simulink model "nms_sim_2D_cost"  (R2024b)
settings: Solver=ode15s  StartTime=0.0  StopTime=t_sim  MaxStep=dt_max  EnableMultiTasking=on
values from neighbouring files (symbols this model uses):
  a_BFSH = param_ctrl(35)*1    [setCtrlPar_optim_CPGreflex2001_2D.m]
  a_GAS = param_ctrl(37)*1    [setCtrlPar_optim_CPGreflex2001_2D.m]
  a_GLU = param_ctrl(31)*1    [setCtrlPar_optim_CPGreflex2001_2D.m]
  a_HAM = param_ctrl(33)*1    [setCtrlPar_optim_CPGreflex2001_2D.m]
  a_HFL = param_ctrl(32)*1    [setCtrlPar_optim_CPGreflex2001_2D.m]
  a_RF = param_ctrl(34)*1    [setCtrlPar_optim_CPGreflex2001_2D.m]
  a_SOL = param_ctrl(38)*1    [setCtrlPar_optim_CPGreflex2001_2D.m]
  a_TA = param_ctrl(39)*1    [setCtrlPar_optim_CPGreflex2001_2D.m]
  a_VAS = param_ctrl(36)*1    [setCtrlPar_optim_CPGreflex2001_2D.m]
  ai = param_ctrl(96)*2.0    [setCtrlPar_optim_CPGreflex2001_2D.m]
  b_BFSH = param_ctrl(52)*.51    [setCtrlPar_optim_CPGreflex2001_2D.m]
  b_BFSHGAS = param_ctrl(55)*.51    [setCtrlPar_optim_CPGreflex2001_2D.m]
  b_BFSHHAM = param_ctrl(54)*.51    [setCtrlPar_optim_CPGreflex2001_2D.m]
  b_BFSHVAS = param_ctrl(53)*.51    [setCtrlPar_optim_CPGreflex2001_2D.m]
  b_GAS = param_ctrl(59)*.51    [setCtrlPar_optim_CPGreflex2001_2D.m]
  b_GASBFSH = param_ctrl(60)*.51    [setCtrlPar_optim_CPGreflex2001_2D.m]
  b_GASSOL = param_ctrl(61)*.51    [setCtrlPar_optim_CPGreflex2001_2D.m]
  b_GLU = param_ctrl(40)*.51    [setCtrlPar_optim_CPGreflex2001_2D.m]
  b_GLUHAM = param_ctrl(42)*.51    [setCtrlPar_optim_CPGreflex2001_2D.m]
  b_GLUHFL = param_ctrl(41)*.51    [setCtrlPar_optim_CPGreflex2001_2D.m]
  b_HAM = param_ctrl(46)*.51    [setCtrlPar_optim_CPGreflex2001_2D.m]
  b_HAMBFSH = param_ctrl(48)*.51    [setCtrlPar_optim_CPGreflex2001_2D.m]
  b_HAMGLU = param_ctrl(47)*.51    [setCtrlPar_optim_CPGreflex2001_2D.m]
  b_HFL = param_ctrl(43)*.51    [setCtrlPar_optim_CPGreflex2001_2D.m]
  b_HFLGLU = param_ctrl(44)*.51    [setCtrlPar_optim_CPGreflex2001_2D.m]
  b_HFLRF = param_ctrl(45)*.51    [setCtrlPar_optim_CPGreflex2001_2D.m]
  b_RF = param_ctrl(49)*.51    [setCtrlPar_optim_CPGreflex2001_2D.m]
  b_RFHFL = param_ctrl(50)*.51    [setCtrlPar_optim_CPGreflex2001_2D.m]
  b_RFVAS = param_ctrl(51)*.51    [setCtrlPar_optim_CPGreflex2001_2D.m]
  b_SOL = param_ctrl(62)*.51    [setCtrlPar_optim_CPGreflex2001_2D.m]
  b_SOLGAS = param_ctrl(64)*.51    [setCtrlPar_optim_CPGreflex2001_2D.m]
  b_SOLTA = param_ctrl(63)*.51    [setCtrlPar_optim_CPGreflex2001_2D.m]
  b_TA = param_ctrl(65)*.51    [setCtrlPar_optim_CPGreflex2001_2D.m]
  b_TASOL = param_ctrl(66)*.51    [setCtrlPar_optim_CPGreflex2001_2D.m]
  b_VAS = param_ctrl(56)*.51    [setCtrlPar_optim_CPGreflex2001_2D.m]
  b_VASBFSH = param_ctrl(57)*.51    [setCtrlPar_optim_CPGreflex2001_2D.m]
  b_VASRF = param_ctrl(58)*.51    [setCtrlPar_optim_CPGreflex2001_2D.m]
  bias = param_ctrl(97)*2.5    [setCtrlPar_optim_CPGreflex2001_2D.m]
  c = 0.05    [nms_MS_2D_scaled.m]
  c_jointstop = 0.3 / (pi/180)    (= 17.1887338539)    [nms_MS_2D_scaled.m]
  D12_F = 0.16    *scaleL_JPhys    [nms_MechInit_2D_scaleSkel.m]
  D12_S = 0.2460	*sub_height    [nms_MechInit_2D_scaleSkel.m]
  D12_T = 0.2450  *sub_height    [nms_MechInit_2D_scaleSkel.m]
  D12y_F = 0.039  *sub_height    [nms_MechInit_2D_scaleSkel.m]
  D12z_HAT = 0.1    [nms_MS_2D_scaled.m]
  D13_F = 0.20    *scaleL_JPhys    [nms_MechInit_2D_scaleSkel.m]
  D1G_F = 0.14    *scaleL_JPhys    [nms_MechInit_2D_scaleSkel.m]
  D1G_HAT = 0.35  *scaleL_JPhys    [nms_MechInit_2D_scaleSkel.m]
  D1G_S = (0.3 - D12y_F/4)	*scaleL_JPhys    [nms_MechInit_2D_scaleSkel.m]
  D1G_T = (0.3 - D12y_F/4)	*scaleL_JPhys    [nms_MechInit_2D_scaleSkel.m]
  D1Gy_F = D12y_F*D1G_F/D12_F    (= 0.07)    [nms_MechInit_2D_scaleSkel.m]
  d_BFSH = param_ctrl(26)*1    [setCtrlPar_optim_CPGreflex2001_2D.m]
  d_GAS = param_ctrl(28)*1    [setCtrlPar_optim_CPGreflex2001_2D.m]
  d_GLU = param_ctrl(22)*1    [setCtrlPar_optim_CPGreflex2001_2D.m]
  d_HAM = param_ctrl(24)*1    [setCtrlPar_optim_CPGreflex2001_2D.m]
  d_HFL = param_ctrl(23)*1    [setCtrlPar_optim_CPGreflex2001_2D.m]
  d_RF = param_ctrl(25)*1    [setCtrlPar_optim_CPGreflex2001_2D.m]
  d_SOL = param_ctrl(29)*1    [setCtrlPar_optim_CPGreflex2001_2D.m]
  d_TA = param_ctrl(30)*1    [setCtrlPar_optim_CPGreflex2001_2D.m]
  d_VAS = param_ctrl(27)*1    [setCtrlPar_optim_CPGreflex2001_2D.m]
  DeltaThRef = 5e-3    (= 0.005)    [nms_MS_2D_scaled.m]
  dloptBFSH = 3.0    (= 3)    [setCtrlPar_optim_CPGreflex2001_2D.m]
  dloptGAS = 3.0    (= 3)    [setCtrlPar_optim_CPGreflex2001_2D.m]
  dloptGLU = 3.0    (= 3)    [setCtrlPar_optim_CPGreflex2001_2D.m]
  dloptHAM = 3.0    (= 3)    [setCtrlPar_optim_CPGreflex2001_2D.m]
  dloptHFL = 3.0    (= 3)    [setCtrlPar_optim_CPGreflex2001_2D.m]
  dloptRF = 3.0    (= 3)    [setCtrlPar_optim_CPGreflex2001_2D.m]
  dloptSOL = 3.0    (= 3)    [setCtrlPar_optim_CPGreflex2001_2D.m]
  dloptTA = 3.0    (= 3)    [setCtrlPar_optim_CPGreflex2001_2D.m]
  dloptVAS = 3.0    (= 3)    [setCtrlPar_optim_CPGreflex2001_2D.m]
  ec_BFSH = param_ctrl(80)*0.15    [setCtrlPar_optim_CPGreflex2001_2D.m]
  ec_GAS = param_ctrl(82)*0.15    [setCtrlPar_optim_CPGreflex2001_2D.m]
  ec_GLU = param_ctrl(76)*0.15    [setCtrlPar_optim_CPGreflex2001_2D.m]
  ec_HAM = param_ctrl(78)*0.15    [setCtrlPar_optim_CPGreflex2001_2D.m]
  ec_HFL = param_ctrl(77)*0.15    [setCtrlPar_optim_CPGreflex2001_2D.m]
  ec_RF = param_ctrl(79)*0.15    [setCtrlPar_optim_CPGreflex2001_2D.m]
  ec_TA = param_ctrl(84)*0.15    [setCtrlPar_optim_CPGreflex2001_2D.m]
  ec_VAS = param_ctrl(81)*0.15    [setCtrlPar_optim_CPGreflex2001_2D.m]
  eref = 0.04    [nms_MS_2D_scaled.m]
  eref_GAS = 0.1    [nms_MS_2D_scaled.m]
  eref_SOL = 0.1    [nms_MS_2D_scaled.m]
  es_BFSH = param_ctrl(89)*0.15    [setCtrlPar_optim_CPGreflex2001_2D.m]
  es_GAS = param_ctrl(91)*0.15    [setCtrlPar_optim_CPGreflex2001_2D.m]
  es_GLU = param_ctrl(85)*0.15    [setCtrlPar_optim_CPGreflex2001_2D.m]
  es_HAM = param_ctrl(87)*0.15    [setCtrlPar_optim_CPGreflex2001_2D.m]
  es_HFL = param_ctrl(86)*0.15    [setCtrlPar_optim_CPGreflex2001_2D.m]
  es_RF = param_ctrl(88)*0.15    [setCtrlPar_optim_CPGreflex2001_2D.m]
  es_TA = param_ctrl(93)*0.15    [setCtrlPar_optim_CPGreflex2001_2D.m]
  es_VAS = param_ctrl(90)*0.15    [setCtrlPar_optim_CPGreflex2001_2D.m]
  FmaxBFSH = 350    [nms_MS_2D_scaled.m]
  FmaxGAS = 2000    [nms_MS_2D_scaled.m]
  FmaxGLU = 4000    [nms_MS_2D_scaled.m]
  FmaxHAM = 2000    [nms_MS_2D_scaled.m]
  FmaxHFL = 2000    [nms_MS_2D_scaled.m]
  FmaxRF = 850    [nms_MS_2D_scaled.m]
  FmaxSOL = 4000    [nms_MS_2D_scaled.m]
  FmaxTA = 800    [nms_MS_2D_scaled.m]
  FmaxVAS = 5000    [nms_MS_2D_scaled.m]
  g = 9.81    [nms_MS_2D_scaled.m]
  gamma_4 = param_ctrl(11) * 1.7    [setCtrlPar_optim_CPGreflexsynergy2023_2D.m]
  h_BFSH = param_ctrl(71)*.1    [setCtrlPar_optim_CPGreflex2001_2D.m]
  h_GAS = param_ctrl(73)*.1    [setCtrlPar_optim_CPGreflex2001_2D.m]
  h_GLU = param_ctrl(67)*.1    [setCtrlPar_optim_CPGreflex2001_2D.m]
  h_HAM = param_ctrl(69)*.1    [setCtrlPar_optim_CPGreflex2001_2D.m]
  h_HFL = param_ctrl(68)*.1    [setCtrlPar_optim_CPGreflex2001_2D.m]
  h_RF = param_ctrl(70)*.1    [setCtrlPar_optim_CPGreflex2001_2D.m]
  h_SOL = param_ctrl(74)*.1    [setCtrlPar_optim_CPGreflex2001_2D.m]
  h_TA = param_ctrl(75)*.1    [setCtrlPar_optim_CPGreflex2001_2D.m]
  h_VAS = param_ctrl(72)*.1    [setCtrlPar_optim_CPGreflex2001_2D.m]
  HLCtrlPar = [theta_tgt l_clr alpha_tgt alpha_cd alpha_cv]    [setCtrlPar_optim_reflex2015_2D.m]
  In_F = 0.005    *scaleM*scaleL_JPhys^2    [nms_MechInit_2D_scaleSkel.m]
  In_HAT = 2.5    *scaleM*scaleL_JPhys^2    [nms_MechInit_2D_scaleSkel.m]
  In_S = 0.05     *scaleM*scaleL_JPhys^2    [nms_MechInit_2D_scaleSkel.m]
  In_T = 0.15     *scaleM*scaleL_JPhys^2    [nms_MechInit_2D_scaleSkel.m]
  init_exc = 0.01    [setInitPar_optim_2D.m]
  init_fm = 0.01    [setInitPar_optim_2D.m]
  init_lce = 1    [setInitPar_optim_2D.m]
  init_LCPG = param_ctrl(12) * 0.01    [setCtrlPar_optim_CPGreflexsynergy2023_2D.m]
  init_LStance = 1    [setInitPar_optim_2D.m]
  init_N1 = osc_signal1(phi_off_osc_ind)    [setCtrlPar_optim_CPGreflex2001_2D.m]
  ... (+441 more)
undefined symbols (not defined in the file or in its folder): cost_act_exponent, cost_v_tgt, flag_controller, Newton, nStep_obj, nStep_startKin, Raphson, sgn, SSW_kin, terrain_slope_angle, v_plateS1, X, Y, Z
libraries: nesl_utility x94, sm_lib x90, simulink x28, simulink_extras x12
(part 3 of 20)

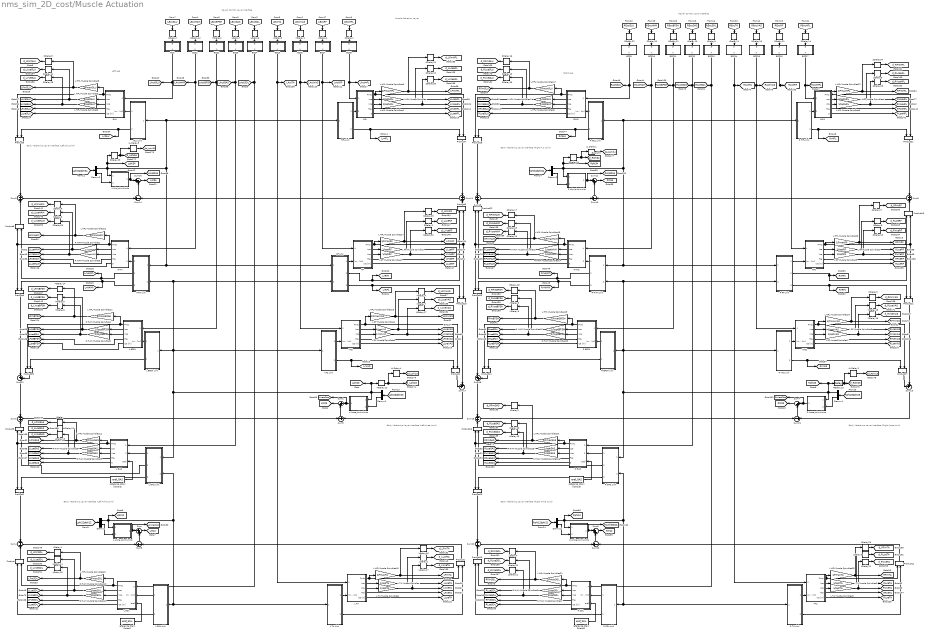
== system nms_sim_2D_cost/Muscle Actuation ==
  note: Left Leg
  note: Neural Control Layer Interface
  note: Muscle Actuation Layer
  note: Body Mechanics Layer
      | Interface (Left Hip Joint)
  note: Body Mechanics Layer
      | Interface (Left Knee Joint)
  note: Body Mechanics Layer
      | Interface (Left Ankle Joint)
  note: Right Leg
  note: Neural Control Layer Interface
  note: Body Mechanics Layer
      | Interface (Right Hip Joint)
  note: Body Mechanics Layer
      | Interface (Right Knee Joint)
  note: Body Mechanics Layer
      | Interface (Right Ankle Joint)
  Demux{,1..5} (6 alike) : Demux  Outputs=2
  ECC : Subsystem
  ECC1 : Subsystem
  ECC10 : Subsystem
  ECC11 : Subsystem
  ECC12 : Subsystem
  ECC13 : Subsystem
  ECC14 : Subsystem
  ECC15 : Subsystem
  ECC16 : Subsystem
  ECC17 : Subsystem
  ECC2 : Subsystem
  ECC3 : Subsystem
  ECC4 : Subsystem
  ECC5 : Subsystem
  ECC6 : Subsystem
  ECC7 : Subsystem
  ECC8 : Subsystem
  ECC9 : Subsystem
  GLU : Subsystem
  GLU Link : Subsystem
  GLU1 : Subsystem
  HAM : Subsystem
  HAM Link : Subsystem
  HAM1 : Subsystem
  HFL : Subsystem
  HFL Link : Subsystem
  HFL1 : Subsystem
  L Ankle Joint Limits : Subsystem
  L BFSH : Subsystem
  L BFSH Link : Subsystem
  L GAS : Subsystem
  L GAS Link : Subsystem
  L HFL Muscle Spindles{,1,4..5} (4 alike) : Gain  Gain=1/loptHFL
  L HFL Muscle Spindles10 : Gain  Gain=1/FmaxHAM
  L HFL Muscle Spindles11 : Gain  Gain=1/FmaxBFSH
  L HFL Muscle Spindles12 : Gain  Gain=1/FmaxGAS
  L HFL Muscle Spindles13 : Gain  Gain=1/FmaxSOL
  L HFL Muscle Spindles14 : Gain  Gain=1/FmaxRF
  L HFL Muscle Spindles15 : Gain  Gain=1/FmaxVAS
  L HFL Muscle Spindles16 : Gain  Gain=1/FmaxTA
  L HFL Muscle Spindles17 : Gain  Gain=1/FmaxGLU
  L HFL Muscle Spindles18 : Gain  Gain=1/FmaxHAM
  L HFL Muscle Spindles19 : Gain  Gain=1/FmaxBFSH
  L HFL Muscle Spindles{2..3,6..7} (4 alike) : Gain  Gain=1/loptGLU
  L HFL Muscle Spindles20 : Gain  Gain=1/FmaxGAS
  L HFL Muscle Spindles21 : Gain  Gain=1/FmaxSOL
  L HFL Muscle Spindles22 : Gain  Gain=1/FmaxHFL
  L HFL Muscle Spindles23 : Gain  Gain=1/FmaxRF
  L HFL Muscle Spindles24 : Gain  Gain=1/FmaxVAS
  L HFL Muscle Spindles25 : Gain  Gain=1/FmaxTA
  L HFL Muscle Spindles8 : Gain  Gain=1/FmaxGLU
  L HFL Muscle Spindles9 : Gain  Gain=1/FmaxHFL
  L Hip Joint Limits : Subsystem
  L Knee Joint Limits : Subsystem
  L RF Muscle Spindles{,1..3} (4 alike) : Gain  Gain=1/loptRF
  L RF Muscle Spindles{4..7} (4 alike) : Gain  Gain=1/loptVAS
  L SOL : Subsystem
  L SOL Link : Subsystem
  L TA : Subsystem
  L TA Muscle Spindles{,1..3} (4 alike) : Gain  Gain=1/loptTA
  L TA Link : Subsystem
  LDelay{,1,3..4,16,23} (6 alike) : TransportDelay  DelayTime=LongDelay  InitialOutput=init_fm
  LDelay{6..11} (6 alike) : TransportDelay  DelayTime=LongDelay  InitialOutput=init_exc
  LDelay{2,5,12,14,18,20} (6 alike) : TransportDelay  DelayTime=LongDelay  InitialOutput=init_lce
  LDelay{13,15,17,19,21..22} (6 alike) : TransportDelay  DelayTime=LongDelay  InitialOutput=init_vce
  LL Delay{1..4} (4 alike) : TransportDelay  DelayTime=LongLoopDelay
  MDelay{1..2,10..11} (4 alike) : TransportDelay  DelayTime=MidDelay  InitialOutput=init_exc
  MDelay12 : TransportDelay  DelayTime=MidDelay  InitialOutput=Lphi230
  MDelay13 : TransportDelay  DelayTime=MidDelay  InitialOutput=Lphi230
  MDelay{3..4,14,18} (4 alike) : TransportDelay  DelayTime=MidDelay  InitialOutput=init_fm
  MDelay{5,7..8,15} (4 alike) : TransportDelay  DelayTime=MidDelay  InitialOutput=init_lce
  MDelay{6,9,16..17} (4 alike) : TransportDelay  DelayTime=MidDelay  InitialOutput=init_vce
  Product{,1..23} (24 alike) : Product  RndMeth=Zero
  R Ankle Joint Limits : Subsystem
  R BFSH : Subsystem
  R BFSH Link : Subsystem
  R GAS : Subsystem
  R GAS Link : Subsystem
  R GLU Link : Subsystem
  R HAM Muscle Spindles{1,3,6,14} (4 alike) : Gain  Gain=1/loptHAM
  R HAM Muscle Spindles{5,7,10..11} (4 alike) : Gain  Gain=1/loptSOL
  R HAM Muscle Spindles{2,4,12..13} (4 alike) : Gain  Gain=1/loptBFSH
  R HAM Muscle Spindles{8..9,15..16} (4 alike) : Gain  Gain=1/loptGAS
  R HAM Link : Subsystem
  R HFL Link : Subsystem
  R Hip Joint Limits : Subsystem
  R Knee Joint Limits : Subsystem
  R RF Link : Subsystem
  R SOL : Subsystem
  R SOL Link : Subsystem
  R TA Link : Subsystem
  R VAS Link : Subsystem
  RF : Subsystem
  RF Link : Subsystem
  RF1 : Subsystem
  SDelay{1,4,7,12,14,20..22} (8 alike) : TransportDelay  DelayTime=ShortDelay  InitialOutput=init_exc
  SDelay{2..3,5..6,10..11,13,15} (8 alike) : TransportDelay  DelayTime=ShortDelay  InitialOutput=init_lce
  SDelay{8..9,16..17,27,29,31,34} (8 alike) : TransportDelay  DelayTime=ShortDelay  InitialOutput=init_fm
  SDelay{18..19,25..26,28,30,32..33} (8 alike) : TransportDelay  DelayTime=ShortDelay  InitialOutput=init_vce
  SDelay23 : TransportDelay  DelayTime=ShortDelay  InitialOutput=Lphi340
  SDelay24 : TransportDelay  DelayTime=ShortDelay  InitialOutput=Lphi340
  Sum{,1,6..7,12,16,18,22} (8 alike) : Sum  Inputs=|++
  Sum{9..10,14,23} (4 alike) : Sum  Inputs=+-
  Sum{2..4,8,11,15,19..20} (8 alike) : Sum
  Sum13 : Sum  Inputs=++|
  Sum17 : Sum  Inputs=++|
  Sum21 : Sum  Inputs=-+
  Sum5 : Sum  Inputs=-+
  TA1 : Subsystem
  VAS : Subsystem
  VAS Link : Subsystem
  VAS1 : Subsystem
  reference strain [lslack] : Constant  Value=eref_SOL
  reference strain [lslack]1 : Constant  Value=eref_SOL
  reference strain [lslack]2 : Constant  Value=eref_GAS
  reference strain [lslack]3 : Constant  Value=eref_GAS
  tag scope: LActBFSH=global, LActGAS=global, LActGLU=global, LActHAM=global, LActHFL=global, LActRF=global, LActSOL=global, LActTA=global, LActVAS=global, LAnkleStop=global, LFceBFSH=global, LFceGAS=global, LFceGLU=global, LFceHAM=global, LFceHFL=global, LFceRF=global, LFceSOL=global, LFceTA=global, LFceVAS=global, LFmBFSH=global, LFmGAS=global, LFmGLU=global, LFmHAM=global, LFmHFL=global, LFmRF=global, LFmSOL=global, LFmTA=global, LFmVAS=global, LHipStop=global, LKneeStop=global, LLceBFSH=global, LLceGAS=global, LLceGLU=global, LLceHAM=global, LLceHFL=global, LLceRF=global, LLceSOL=global, LLceTA=global, LLceVAS=global, LLseBFSH=global, LLseGAS=global, LLseGLU=global, LLseHAM=global, LLseHFL=global, LLseRF=global, LLseSOL=global, LLseTA=global, LLseVAS=global, LM12=global, LM23=global, LM34=global, LVceBFSH=global, LVceGAS=global, LVceGLU=global, LVceHAM=global, LVceHFL=global, LVceRF=global, LVceSOL=global, LVceTA=global, LVceVAS=global, Lphi12=global, Lphi23=global, Lphi34=global, LrGLU=global, LrHAMh=global, LrHAMk=global, LrHFL=global, LrRFh=global, LrRFk=global, LrVAS=global, RActBFSH=global, RActGAS=global, RActGLU=global, RActHAM=global, RActHFL=global, RActRF=global, RActSOL=global, RActTA=global, RActVAS=global, RAnkleStop=global, RFceBFSH=global, RFceGAS=global, RFceGLU=global, RFceHAM=global, RFceHFL=global, RFceRF=global, RFceSOL=global, RFceTA=global, RFceVAS=global, RFmBFSH=global, RFmGAS=global, RFmGLU=global, RFmHAM=global, RFmHFL=global, RFmRF=global, RFmSOL=global, RFmTA=global, RFmVAS=global, RHipStop=global, RKneeStop=global, RLceBFSH=global, RLceGAS=global, RLceGLU=global, RLceHAM=global, RLceHFL=global, RLceRF=global, RLceSOL=global, RLceTA=global, RLceVAS=global, RLseBFSH=global, RLseGAS=global, RLseGLU=global, RLseHAM=global, RLseHFL=global, RLseRF=global, RLseSOL=global, RLseTA=global, RLseVAS=global, RM12=global, RM23=global, RM34=global, RVceBFSH=global, RVceGAS=global, RVceGLU=global, RVceHAM=global, RVceHFL=global, RVceRF=global, RVceSOL=global, RVceTA=global, RVceVAS=global, Rphi12=global, Rphi23=global, Rphi34=global, RrGLU=global, RrHAMh=global, RrHAMk=global, RrHFL=global, RrRFh=global, RrRFk=global, RrVAS=global, d_LFmBFSH=global, d_LFmGAS=global, d_LFmGLU=global, d_LFmHAM=global, d_LFmHFL=global, d_LFmRF=global, d_LFmSOL=global, d_LFmTA=global, d_LFmVAS=global, d_LLceBFSH=global, d_LLceGAS=global, d_LLceGLU=global, d_LLceHAM=global, d_LLceHFL=global, d_LLceRF=global, d_LLceSOL=global, d_LLceTA=global, d_LLceVAS=global, d_LVceBFSH=global, d_LVceGAS=global, d_LVceGLU=global, d_LVceHAM=global, d_LVceHFL=global, d_LVceRF=global, d_LVceSOL=global, d_LVceTA=global, d_LVceVAS=global, d_Lphi23=global, d_Lphi34=global, d_RFmBFSH=global, d_RFmGAS=global, d_RFmGLU=global, d_RFmHAM=global, d_RFmHFL=global, d_RFmRF=global, d_RFmSOL=global, d_RFmTA=global, d_RFmVAS=global, d_RLceBFSH=global, d_RLceGAS=global, d_RLceGLU=global, d_RLceHAM=global, d_RLceHFL=global, d_RLceRF=global, d_RLceSOL=global, d_RLceTA=global, d_RLceVAS=global, d_RVceBFSH=global, d_RVceGAS=global, d_RVceGLU=global, d_RVceHAM=global, d_RVceHFL=global, d_RVceRF=global, d_RVceSOL=global, d_RVceTA=global, d_RVceVAS=global, d_Rphi23=global, d_Rphi34=global, dd_Lphi23=global, dd_Lphi34=global, dd_Rphi23=global, dd_Rphi34=global
  wires:
  Demux1/1 -> L Knee Joint Limits/1(phi [rad]), L BFSH Link/1(phi23 [rad]), HAM Link/2(phi23 [rad]), RF Link/2(phi23 [rad]), VAS Link/1(phi23 [rad]), L GAS Link/1(phi23 [rad]), MDelay12/1, [Lphi23]
  L SOL/1(Fmtc) -> L HFL Muscle Spindles13/1, Product/2
  L TA/2(Lce) -> L TA Muscle Spindles/1
  L GAS/1(Fmtc) -> Product2/1, Product3/1, L HFL Muscle Spindles12/1
  Demux/1 -> L SOL Link/1(phi12 [rad]), L TA Link/1(phi12 [rad]), L GAS Link/2(phi12 [rad]), L Ankle Joint Limits/1(phi [rad]), [Lphi12]
  HAM/1(Fmtc) -> Product9/1, Product8/1, L HFL Muscle Spindles10/1
  HAM/2(Lce) -> R HAM Muscle Spindles1/1
  HFL/1(Fmtc) -> L HFL Muscle Spindles9/1, Product7/2
  HFL/2(Lce) -> L HFL Muscle Spindles/1
  GLU/1(Fmtc) -> Product6/1, L HFL Muscle Spindles8/1
  Sum16/1 -> [LM34]
  Demux/2 -> L Ankle Joint Limits/2(dphi [rad/s])
  Sum9/1 -> Sum/2
  Demux1/2 -> L Knee Joint Limits/2(dphi [rad/s])
  L SOL Link/1(lmtc [m]) -> L SOL/2(lmtc [m])
  L TA Link/1(lmtc [m]) -> L TA/2(lmtc [m])
  L GAS Link/3(lever12 [m]) -> Product2/2
  L GAS Link/2(lever23 [m]) -> Product3/2
  L GAS Link/1(lmtu [m]) -> L GAS/2(lmtc [m])
  VAS Link/1(lmtu [m]) -> VAS/2(lmtc [m])
  HAM Link/1(lmtu [m]) -> HAM/2(lmtc [m])
  HAM Link/2(lever34 [m]) -> Product8/2, [LrHAMh]
  HAM Link/3(lever23 [m]) -> Product9/2, [LrHAMk]
  Product3/1 -> Sum2/2
  Sum3/1 -> Sum14/1
  Sum4/1 -> Sum9/1
  [Lphi12dphi12] -> Demux/1
  [Lphi23dphi23] -> Demux1/1
  [Lphi34dphi34] -> Demux2/1
  Demux2/1 -> L Hip Joint Limits/1(phi [rad]), HFL Link/1(phi34 [rad]), GLU Link/1(phi34 [rad]), RF Link/1(phi34 [rad]), HAM Link/1(phi34 [rad]), [Lphi34], SDelay23/1
  L SOL Link/2(lever [m]) -> Product/1
  Product/1 -> Sum4/2
  Product2/1 -> Sum4/1
  L TA Link/2(lever [m]) -> Product1/2
  Product1/1 -> Sum9/2
  L Ankle Joint Limits/1(M_stop [Nm]) -> Sum/1, [LAnkleStop]
  Sum/1 -> [LM12]
  VAS/1(Fmtc) -> Product4/2, L HFL Muscle Spindles15/1
  Sum1/1 -> [LM23]
  L Knee Joint Limits/1(M_stop [Nm]) -> Sum1/1, [LKneeStop]
  Sum5/1 -> Sum1/2
  VAS Link/2(lever [m]) -> [LrVAS], Product4/1
  Sum2/1 -> Sum5/1
  Product8/1 -> Sum3/2
  Product6/1 -> Sum3/1
  GLU Link/1(lmtu [m]) -> GLU/2(lmtc [m])
  GLU Link/2(lever [m]) -> [LrGLU], Product6/2
  Demux2/2 -> L Hip Joint Limits/2(dphi [rad/s])
  L Hip Joint Limits/1(M_stop [Nm]) -> Sum16/1, [LHipStop]
  Sum14/1 -> Sum16/2
  HFL Link/1(lmtu [m]) -> HFL/2(lmtc [m])
  HFL Link/2(lever [m]) -> Product7/1, [LrHFL]
  GLU/2(Lce) -> L HFL Muscle Spindles3/1
  GLU/3(Vce) -> L HFL Muscle Spindles2/1
  HAM/3(Vce) -> R HAM Muscle Spindles6/1
  L GAS/3(Vce) -> R HAM Muscle Spindles9/1
  L GAS/2(Lce) -> R HAM Muscle Spindles8/1
  L SOL/2(Lce) -> R HAM Muscle Spindles10/1
  L SOL/3(Vce) -> R HAM Muscle Spindles11/1
  L TA/3(Vce) -> L TA Muscle Spindles1/1
  VAS/3(Vce) -> L RF Muscle Spindles6/1
  VAS/2(Lce) -> L RF Muscle Spindles4/1
  HFL/3(Vce) -> L HFL Muscle Spindles1/1
  RF/3(Vce) -> L RF Muscle Spindles2/1
  RF/2(Lce) -> L RF Muscle Spindles/1
  RF Link/1(lmtu [m]) -> RF/2(lmtc [m])
  RF Link/2(lever34 [m]) -> Product5/1, [LrRFh]
  RF Link/3(lever23 [m]) -> Product15/1, [LrRFk]
  Product7/1 -> Sum11/1
  Product5/1 -> Sum11/2
  Product15/1 -> Sum17/2
  Sum17/1 -> Sum5/2
  Product4/1 -> Sum17/1
  L BFSH Link/1(lmtu [m]) -> L BFSH/2(lmtc [m])
  L BFSH Link/2(lever [m]) -> Product20/2
  L BFSH/2(Lce) -> R HAM Muscle Spindles4/1
  L BFSH/3(Vce) -> R HAM Muscle Spindles2/1
  Product20/1 -> Sum22/2
  Sum22/1 -> Sum2/1
  Product9/1 -> Sum22/1
  L HFL Muscle Spindles1/1 -> SDelay30/1, [LVceHFL]
  L HFL Muscle Spindles2/1 -> SDelay25/1, [LVceGLU]
  L HFL Muscle Spindles3/1 -> SDelay11/1, [LLceGLU]
  L RF Muscle Spindles6/1 -> [LVceVAS], MDelay17/1
  RF/1(Fmtc) -> Product15/2, Product5/2, L HFL Muscle Spindles14/1
  L BFSH/1(Fmtc) -> Product20/1, L HFL Muscle Spindles11/1
  R HAM Muscle Spindles8/1 -> LDelay12/1, [LLceGAS]
  R HAM Muscle Spindles9/1 -> LDelay13/1, [LVceGAS]
  R HAM Muscle Spindles10/1 -> LDelay14/1, [LLceSOL]
  R HAM Muscle Spindles11/1 -> LDelay15/1, [LVceSOL]
  L TA/1(Fmtc) -> Product1/1, L HFL Muscle Spindles16/1
  L TA Muscle Spindles1/1 -> LDelay17/1, [LVceTA]
  L HFL Muscle Spindles/1 -> SDelay10/1, [LLceHFL]
  R HAM Muscle Spindles1/1 -> SDelay3/1, [LLceHAM]
  R HAM Muscle Spindles6/1 -> SDelay33/1, [LVceHAM]
  L RF Muscle Spindles/1 -> SDelay2/1, [LLceRF]
  L RF Muscle Spindles2/1 -> SDelay32/1, [LVceRF]
  R HAM Muscle Spindles4/1 -> MDelay5/1, [LLceBFSH]
  R HAM Muscle Spindles2/1 -> MDelay6/1, [LVceBFSH]
  L RF Muscle Spindles4/1 -> [LLceVAS], MDelay7/1
  L TA Muscle Spindles/1 -> [LLceTA], LDelay2/1
  Demux4/1 -> R Knee Joint Limits/1(phi [rad]), R VAS Link/1(phi23 [rad]), R RF Link/2(phi23 [rad]), R HAM Link/2(phi23 [rad]), R BFSH Link/1(phi23 [rad]), R GAS Link/1(phi23 [rad]), MDelay13/1, [Rphi23]
  R SOL/1(Fmtc) -> Product10/2, L HFL Muscle Spindles21/1
  TA1/2(Lce) -> L TA Muscle Spindles2/1
  R GAS/1(Fmtc) -> Product13/1, Product16/1, L HFL Muscle Spindles20/1
  Demux3/1 -> R SOL Link/1(phi12 [rad]), R TA Link/1(phi12 [rad]), R GAS Link/2(phi12 [rad]), R Ankle Joint Limits/1(phi [rad]), [Rphi12]
  HAM1/1(Fmtc) -> Product23/1, Product22/1, L HFL Muscle Spindles18/1
  HAM1/2(Lce) -> R HAM Muscle Spindles3/1
  HFL1/1(Fmtc) -> L HFL Muscle Spindles22/1, Product21/2
  HFL1/2(Lce) -> L HFL Muscle Spindles4/1
  GLU1/1(Fmtc) -> Product19/1, L HFL Muscle Spindles17/1
  Sum12/1 -> [RM34]
  Demux3/2 -> R Ankle Joint Limits/2(dphi [rad/s])
  Sum23/1 -> Sum6/2
  Demux4/2 -> R Knee Joint Limits/2(dphi [rad/s])
  R SOL Link/1(lmtc [m]) -> R SOL/2(lmtc [m])
  R TA Link/1(lmtc [m]) -> TA1/2(lmtc [m])
  R GAS Link/3(lever12 [m]) -> Product13/2
  R GAS Link/2(lever23 [m]) -> Product16/2
  R GAS Link/1(lmtu [m]) -> R GAS/2(lmtc [m])
  R HAM Link/1(lmtu [m]) -> HAM1/2(lmtc [m])
  R HAM Link/2(lever34 [m]) -> Product22/2, [RrHAMh]
  R HAM Link/3(lever23 [m]) -> Product23/2, [RrHAMk]
  Product16/1 -> Sum15/2
  Sum19/1 -> Sum10/1
  Sum20/1 -> Sum23/1
  [Rphi12dphi12] -> Demux3/1
  [Rphi23dphi23] -> Demux4/1
  [Rphi34dphi34] -> Demux5/1
  Demux5/1 -> R Hip Joint Limits/1(phi [rad]), R HFL Link/1(phi34 [rad]), R GLU Link/1(phi34 [rad]), R RF Link/1(phi34 [rad]), R HAM Link/1(phi34 [rad]), SDelay24/1, [Rphi34]
  R SOL Link/2(lever [m]) -> Product10/1
  Product10/1 -> Sum20/2
  Product13/1 -> Sum20/1
  R TA Link/2(lever [m]) -> Product11/2
  Product11/1 -> Sum23/2
  R Ankle Joint Limits/1(M_stop [Nm]) -> Sum6/1, [RAnkleStop]
  Sum6/1 -> [RM12]
  VAS1/1(Fmtc) -> Product17/2, L HFL Muscle Spindles24/1
  Sum7/1 -> [RM23]
  R Knee Joint Limits/1(M_stop [Nm]) -> Sum7/1, [RKneeStop]
  Sum21/1 -> Sum7/2
  R VAS Link/2(lever [m]) -> [RrVAS], Product17/1
  Sum15/1 -> Sum21/1
  Product22/1 -> Sum19/2
  Product19/1 -> Sum19/1
  R GLU Link/1(lmtu [m]) -> GLU1/2(lmtc [m])
  R GLU Link/2(lever [m]) -> Product19/2, [RrGLU]
  Demux5/2 -> R Hip Joint Limits/2(dphi [rad/s])
  R Hip Joint Limits/1(M_stop [Nm]) -> [RHipStop], Sum12/1
  Sum10/1 -> Sum12/2
  R HFL Link/1(lmtu [m]) -> HFL1/2(lmtc [m])
  R HFL Link/2(lever [m]) -> Product21/1, [RrHFL]
  GLU1/2(Lce) -> L HFL Muscle Spindles7/1
  GLU1/3(Vce) -> L HFL Muscle Spindles6/1
  HAM1/3(Vce) -> R HAM Muscle Spindles14/1
  R GAS/3(Vce) -> R HAM Muscle Spindles16/1
  R GAS/2(Lce) -> R HAM Muscle Spindles15/1
  R SOL/2(Lce) -> R HAM Muscle Spindles5/1
  R SOL/3(Vce) -> R HAM Muscle Spindles7/1
  TA1/3(Vce) -> L TA Muscle Spindles3/1
  VAS1/3(Vce) -> L RF Muscle Spindles7/1
  VAS1/2(Lce) -> L RF Muscle Spindles5/1
  HFL1/3(Vce) -> L HFL Muscle Spindles5/1
  RF1/3(Vce) -> L RF Muscle Spindles3/1
  RF1/2(Lce) -> L RF Muscle Spindles1/1
  R RF Link/2(lever34 [m]) -> Product18/1, [RrRFh]
  R RF Link/3(lever23 [m]) -> Product12/1, [RrRFk]
  Sum8/1 -> Sum10/2
  Product21/1 -> Sum8/1
  Product18/1 -> Sum8/2
  Product12/1 -> Sum13/2
  Sum13/1 -> Sum21/2
  Product17/1 -> Sum13/1
  R BFSH Link/1(lmtu [m]) -> R BFSH/2(lmtc [m])
  R BFSH Link/2(lever [m]) -> Product14/2
  R BFSH/2(Lce) -> R HAM Muscle Spindles13/1
  R BFSH/3(Vce) -> R HAM Muscle Spindles12/1
  Product14/1 -> Sum18/2
  Sum18/1 -> Sum15/1
  Product23/1 -> Sum18/1
  L HFL Muscle Spindles5/1 -> [RVceHFL], SDelay28/1
  L HFL Muscle Spindles6/1 -> SDelay26/1, [RVceGLU]
  L HFL Muscle Spindles7/1 -> SDelay13/1, [RLceGLU]
  RF1/1(Fmtc) -> Product18/2, Product12/2, L HFL Muscle Spindles23/1
  R BFSH/1(Fmtc) -> Product14/1, L HFL Muscle Spindles19/1
  R HAM Muscle Spindles15/1 -> LDelay18/1, [RLceGAS]
  R HAM Muscle Spindles16/1 -> LDelay19/1, [RVceGAS]
  R HAM Muscle Spindles5/1 -> LDelay20/1, [RLceSOL]
  R HAM Muscle Spindles7/1 -> LDelay21/1, [RVceSOL]
  TA1/1(Fmtc) -> Product11/1, L HFL Muscle Spindles25/1
  L TA Muscle Spindles3/1 -> [RVceTA], LDelay22/1
  L HFL Muscle Spindles4/1 -> [RLceHFL], SDelay6/1
  R HAM Muscle Spindles3/1 -> SDelay15/1, [RLceHAM]
  R HAM Muscle Spindles14/1 -> SDelay19/1, [RVceHAM]
  L RF Muscle Spindles1/1 -> SDelay5/1, [RLceRF]
  L RF Muscle Spindles3/1 -> SDelay18/1, [RVceRF]
  R HAM Muscle Spindles13/1 -> MDelay8/1, [RLceBFSH]
  R HAM Muscle Spindles12/1 -> MDelay9/1, [RVceBFSH]
  L RF Muscle Spindles5/1 -> MDelay15/1, [RLceVAS]
  L TA Muscle Spindles2/1 -> [RLceTA], LDelay5/1
  R VAS Link/1(lmtu [m]) -> VAS1/2(lmtc [m])
  R RF Link/1(lmtu [m]) -> RF1/2(lmtc [m])
  ECC/1(A) -> GLU/1(A), [LActGLU]
  GLU/4(Fce) -> [LFceGLU]
  GLU/5(lse [m]) -> [LLseGLU]
  L HFL Muscle Spindles10/1 -> SDelay9/1, [LFmHAM]
  ECC1/1(A) -> [LActHAM], HAM/1(A)
  HAM/4(Fce) -> [LFceHAM]
  HAM/5(lse [m]) -> [LLseHAM]
  L HFL Muscle Spindles11/1 -> MDelay14/1, [LFmBFSH]
  ECC2/1(A) -> [LActBFSH], L BFSH/1(A)
  L BFSH/4(Fce) -> [LFceBFSH]
  L BFSH/5(lse [m]) -> [LLseBFSH]
  ECC3/1(A) -> [LActGAS], L GAS/1(A)
  ECC4/1(A) -> L SOL/1(A), [LActSOL]
  ECC5/1(A) -> [LActTA], L TA/1(A)
  ECC6/1(A) -> [LActVAS], VAS/1(A)
  ECC7/1(A) -> [LActRF], RF/1(A)
  ECC8/1(A) -> HFL/1(A), [LActHFL]
  L GAS/4(Fce) -> [LFceGAS]
  L GAS/5(lse [m]) -> [LLseGAS]
  L HFL Muscle Spindles12/1 -> LDelay/1, [LFmGAS]
  L HFL Muscle Spindles13/1 -> LDelay1/1, [LFmSOL]
  L SOL/4(Fce) -> [LFceSOL]
  L SOL/5(lse [m]) -> [LLseSOL]
  L HFL Muscle Spindles16/1 -> LDelay16/1, [LFmTA]
  L TA/4(Fce) -> [LFceTA]
  L TA/5(lse [m]) -> [LLseTA]
  L HFL Muscle Spindles15/1 -> [LFmVAS], MDelay4/1
  VAS/4(Fce) -> [LFceVAS]
  VAS/5(lse [m]) -> [LLseVAS]
  L HFL Muscle Spindles14/1 -> SDelay29/1, [LFmRF]
  RF/4(Fce) -> [LFceRF]
  RF/5(lse [m]) -> [LLseRF]
  L HFL Muscle Spindles9/1 -> SDelay31/1, [LFmHFL]
  HFL/4(Fce) -> [LFceHFL]
  HFL/5(lse [m]) -> [LLseHFL]
  ECC9/1(A) -> [RActGLU], GLU1/1(A)
  ECC10/1(A) -> [RActHAM], HAM1/1(A)
  ECC11/1(A) -> [RActBFSH], R BFSH/1(A)
  ECC12/1(A) -> R GAS/1(A), [RActGAS]
  ECC13/1(A) -> R SOL/1(A), [RActSOL]
  ECC14/1(A) -> [RActTA], TA1/1(A)
  ECC15/1(A) -> [RActVAS], VAS1/1(A)
  ECC16/1(A) -> [RActRF], RF1/1(A)
  ECC17/1(A) -> HFL1/1(A), [RActHFL]
  L HFL Muscle Spindles17/1 -> SDelay16/1, [RFmGLU]
  GLU1/5(lse [m]) -> [RLseGLU]
  L HFL Muscle Spindles18/1 -> SDelay17/1, [RFmHAM]
  HAM1/4(Fce) -> [RFceHAM]
  HAM1/5(lse [m]) -> [RLseHAM]
  L HFL Muscle Spindles19/1 -> MDelay18/1, [RFmBFSH]
  R BFSH/4(Fce) -> [RFceBFSH]
  R BFSH/5(lse [m]) -> [RLseBFSH]
  L HFL Muscle Spindles20/1 -> LDelay3/1, [RFmGAS]
  R GAS/4(Fce) -> [RFceGAS]
  R GAS/5(lse [m]) -> [RLseGAS]
  L HFL Muscle Spindles21/1 -> LDelay4/1, [RFmSOL]
  R SOL/4(Fce) -> [RFceSOL]
  R SOL/5(lse [m]) -> [RLseSOL]
  L HFL Muscle Spindles25/1 -> LDelay23/1, [RFmTA]
  TA1/4(Fce) -> [RFceTA]
  TA1/5(lse [m]) -> [RLseTA]
  L HFL Muscle Spindles24/1 -> [RFmVAS], MDelay3/1
  VAS1/4(Fce) -> [RFceVAS]
  VAS1/5(lse [m]) -> [RLseVAS]
  L HFL Muscle Spindles23/1 -> SDelay27/1, [RFmRF]
  RF1/4(Fce) -> [RFceRF]
  RF1/5(lse [m]) -> [RLseRF]
  L HFL Muscle Spindles22/1 -> SDelay34/1, [RFmHFL]
  HFL1/4(Fce) -> [RFceHFL]
  HFL1/5(lse [m]) -> [RLseHFL]
  reference strain [lslack]/1 -> L SOL/3(eref)
  reference strain [lslack]1/1 -> R SOL/3(eref)
  reference strain [lslack]2/1 -> L GAS/3(eref)
  reference strain [lslack]3/1 -> R GAS/3(eref)
  SDelay8/1 -> [d_LFmGLU]
  L HFL Muscle Spindles8/1 -> SDelay8/1, [LFmGLU]
  SDelay9/1 -> [d_LFmHAM]
  MDelay4/1 -> [d_LFmVAS]
  MDelay5/1 -> [d_LLceBFSH]
  LDelay/1 -> [d_LFmGAS]
  LDelay1/1 -> [d_LFmSOL]
  LDelay2/1 -> [d_LLceTA]
  SDelay2/1 -> [d_LLceRF]
  SDelay32/1 -> [d_LVceRF]
  SDelay3/1 -> [d_LLceHAM]
  SDelay33/1 -> [d_LVceHAM]
  MDelay17/1 -> [d_LVceVAS]
  MDelay6/1 -> [d_LVceBFSH]
  SDelay10/1 -> [d_LLceHFL]
  SDelay11/1 -> [d_LLceGLU]
  MDelay7/1 -> [d_LLceVAS]
  SDelay16/1 -> [d_RFmGLU]
  SDelay17/1 -> [d_RFmHAM]
  MDelay3/1 -> [d_RFmVAS]
  MDelay8/1 -> [d_RLceBFSH]
  LDelay3/1 -> [d_RFmGAS]
  LDelay4/1 -> [d_RFmSOL]
  LDelay5/1 -> [d_RLceTA]
  SDelay5/1 -> [d_RLceRF]
  SDelay18/1 -> [d_RVceRF]
  SDelay15/1 -> [d_RLceHAM]
  SDelay19/1 -> [d_RVceHAM]
  MDelay16/1 -> [d_RVceVAS]
  L RF Muscle Spindles7/1 -> MDelay16/1, [RVceVAS]
  MDelay9/1 -> [d_RVceBFSH]
  SDelay6/1 -> [d_RLceHFL]
  SDelay13/1 -> [d_RLceGLU]
  MDelay15/1 -> [d_RLceVAS]
  MDelay1/1 -> ECC6/1(E)
  LDelay6/1 -> ECC4/1(E)
  [LExcGAS] -> LDelay7/1
  LDelay7/1 -> ECC3/1(E)
  [LExcVAS] -> MDelay1/1
  [LExcSOL] -> LDelay6/1
  LDelay8/1 -> ECC5/1(E)
  SDelay12/1 -> ECC1/1(E)
  [LExcHAM] -> SDelay12/1
  SDelay4/1 -> ECC7/1(E)
  [LExcTA] -> LDelay8/1
  SDelay1/1 -> ECC8/1(E)
  [LExcRF] -> SDelay4/1
  [LExcHFL] -> SDelay1/1
  MDelay2/1 -> ECC2/1(E)
  SDelay7/1 -> ECC/1(E)
  [LExcBFSH] -> MDelay2/1
  [LExcGLU] -> SDelay7/1
  [RExcGAS] -> LDelay10/1
  [RExcVAS] -> MDelay10/1
  [RExcSOL] -> LDelay9/1
  [RExcHAM] -> SDelay20/1
  [RExcTA] -> LDelay11/1
  [RExcRF] -> SDelay21/1
  [RExcHFL] -> SDelay14/1
  [RExcBFSH] -> MDelay11/1
  [RExcGLU] -> SDelay22/1
  Sum11/1 -> Sum14/2
  SDelay23/1 -> LL Delay3/1, [d_Lphi34]
  MDelay12/1 -> LL Delay4/1, [d_Lphi23]
  MDelay13/1 -> LL Delay2/1, [d_Rphi23]
  LL Delay3/1 -> [dd_Lphi34]
  LL Delay1/1 -> [dd_Rphi34]
  SDelay24/1 -> LL Delay1/1, [d_Rphi34]
  LL Delay2/1 -> [dd_Rphi23]
  LL Delay4/1 -> [dd_Lphi23]
  SDelay25/1 -> [d_LVceGLU]
  MDelay14/1 -> [d_LFmBFSH]
  LDelay13/1 -> [d_LVceGAS]
  LDelay12/1 -> [d_LLceGAS]
  LDelay15/1 -> [d_LVceSOL]
  LDelay14/1 -> [d_LLceSOL]
  LDelay17/1 -> [d_LVceTA]
  LDelay16/1 -> [d_LFmTA]
  SDelay29/1 -> [d_LFmRF]
  SDelay31/1 -> [d_LFmHFL]
  SDelay30/1 -> [d_LVceHFL]
  SDelay26/1 -> [d_RVceGLU]
  GLU1/4(Fce) -> [RFceGLU]
  MDelay18/1 -> [d_RFmBFSH]
  LDelay19/1 -> [d_RVceGAS]
  LDelay18/1 -> [d_RLceGAS]
  LDelay20/1 -> [d_RLceSOL]
  LDelay21/1 -> [d_RVceSOL]
  LDelay22/1 -> [d_RVceTA]
  LDelay23/1 -> [d_RFmTA]
  SDelay27/1 -> [d_RFmRF]
  SDelay28/1 -> [d_RVceHFL]
  SDelay34/1 -> [d_RFmHFL]
  SDelay21/1 -> ECC16/1(E)
  SDelay14/1 -> ECC17/1(E)
  LDelay10/1 -> ECC12/1(E)
  MDelay10/1 -> ECC15/1(E)
  SDelay20/1 -> ECC10/1(E)
  SDelay22/1 -> ECC9/1(E)
  MDelay11/1 -> ECC11/1(E)
  LDelay9/1 -> ECC13/1(E)
  LDelay11/1 -> ECC14/1(E)

== system nms_sim_2D_cost/Muscle synergy Controller ==
  note: Movement Generator
  note: Movement Regulator
  From Workspace : FromWorkspace  VariableName=pulse1L
  From Workspace1 : FromWorkspace  VariableName=pulse2L
  From Workspace2 : FromWorkspace  VariableName=pulse3L
  From Workspace3 : FromWorkspace  VariableName=pulse4L
  From Workspace4 : FromWorkspace  VariableName=pulse5L
  From Workspace5 : FromWorkspace  VariableName=pulse1R
  From Workspace6 : FromWorkspace  VariableName=pulse2R
  From Workspace7 : FromWorkspace  VariableName=pulse3R
  From Workspace8 : FromWorkspace  VariableName=pulse4R
  From Workspace9 : FromWorkspace  VariableName=pulse5R
  LL Delay{1..8} (8 alike) : TransportDelay  DelayTime=LongLoopDelay
  Left Movement Generator : Subsystem
  Left Movement Regulator : Subsystem
  Mux : Mux  Inputs=9
  Mux1 : Mux  Inputs=9
  Right Movement Generator : Subsystem
  Right Movement Regulator : Subsystem
  Saturation1 : Saturate  UpperLimit=1  LowerLimit=0.01
  Saturation18 : Saturate  UpperLimit=1  LowerLimit=0.01
  Selector : Selector  InputPortWidth=3  IndexOptions=Index vector (dialog)  Indices=1  OutputSizes=1
  Selector1 : Selector  InputPortWidth=3  IndexOptions=Index vector (dialog)  Indices=1  OutputSizes=1
  Sum{,1..7} (8 alike) : Sum
  LExc : Outport
  RExc : Outport  Port=2
  wires:
  Left Movement Regulator/1(LExcHFL_MR) -> LL Delay3/1  "LHFL"
  Left Movement Regulator/2(LExcGLU_MR) -> LL Delay1/1  "LGLU"
  Left Movement Regulator/3(LExcTA_MR) -> LL Delay2/1  "LTA"
  Left Movement Regulator/4(LExcSOL_MR) -> LL Delay4/1  "LSOL"
  [d_dtheta] -> Left Movement Regulator/2(dtheta)
  [dd_dxyzHAT] -> Selector/1
  [d_dtheta] -> Right Movement Regulator/2(dtheta)
  [dd_dxyzHAT] -> Selector1/1
  [d_theta] -> Right Movement Regulator/1(theta)
  Right Movement Regulator/2(RExcGLU_MR) -> LL Delay5/1  "RGLU"
  Right Movement Regulator/1(RExcHFL_MR) -> LL Delay7/1  "RHFL"
  Right Movement Regulator/4(RExcSOL_MR) -> LL Delay8/1  "RSOL"
  Right Movement Regulator/3(RExcTA_MR) -> LL Delay6/1  "RTA"
  LL Delay3/1 -> [LExcHFL_MR]
  LL Delay1/1 -> [LExcGLU_MR]
  LL Delay2/1 -> [LExcTA_MR]
  LL Delay4/1 -> [LExcSOL_MR]
  LL Delay7/1 -> [RExcHFL_MR]
  LL Delay5/1 -> [RExcGLU_MR]
  LL Delay6/1 -> [RExcTA_MR]
  LL Delay8/1 -> [RExcSOL_MR]
  [d_theta] -> Left Movement Regulator/1(theta)
  Selector/1 -> Left Movement Regulator/3(v)
  Selector1/1 -> Right Movement Regulator/3(v)
  [d_RStance] -> Right Movement Regulator/4(Stance)
  [d_LStance] -> Left Movement Regulator/4(Stance)
  From Workspace/1 -> Left Movement Generator/1(P1)
  Left Movement Generator/9(TA) -> [LExcTA_MG]
  From Workspace9/1 -> Right Movement Generator/5(P5)
  Right Movement Generator/3(HAM) -> [RExcHAM_MG]
  From Workspace5/1 -> Right Movement Generator/1(P1)
  From Workspace3/1 -> Left Movement Generator/4(P4)
  Left Movement Generator/8(SOL) -> [LExcSOL_MG]
  Right Movement Generator/2(GLU) -> [RExcGLU_MG]
  Left Movement Generator/6(BFSH) -> [LExcBFSH_MG]
  Right Movement Generator/9(TA) -> [RExcTA_MG]
  Left Movement Generator/4(VAS) -> [LExcVAS_MG]
  Left Movement Generator/2(GLU) -> [LExcGLU_MG]
  Right Movement Generator/8(SOL) -> [RExcSOL_MG]
  Left Movement Generator/3(HAM) -> [LExcHAM_MG]
  Left Movement Generator/7(GAS) -> [LExcGAS_MG]
  Right Movement Generator/7(GAS) -> [RExcGAS_MG]
  Right Movement Generator/6(BFSH) -> [RExcBFSH_MG]
  From Workspace1/1 -> Left Movement Generator/2(P2)
  Right Movement Generator/5(RF) -> [RExcRF_MG]
  From Workspace6/1 -> Right Movement Generator/2(P2)
  From Workspace4/1 -> Left Movement Generator/5(P5)
  Right Movement Generator/4(VAS) -> [RExcVAS_MG]
  From Workspace7/1 -> Right Movement Generator/3(P3)
  From Workspace8/1 -> Right Movement Generator/4(P4)
  Left Movement Generator/5(RF) -> [LExcRF_MG]
  Right Movement Generator/1(HFL) -> [RExcHFL_MG]
  From Workspace2/1 -> Left Movement Generator/3(P3)
  Left Movement Generator/1(HFL) -> [LExcHFL_MG]
  Sum6/1 -> Mux1/9
  [LExcBFSH_MG] -> Mux/6
  [LExcGLU_MR] -> Sum1/1
  [LExcHAM_MG] -> Mux/3
  Sum2/1 -> Mux/9
  [RExcGLU_MG] -> Sum5/2
  [RExcHAM_MG] -> Mux1/3
  [RExcBFSH_MG] -> Mux1/6
  [LExcVAS_MG] -> Mux/5
  Sum5/1 -> Mux1/2
  [RExcTA_MR] -> Sum6/1
  [LExcHFL_MR] -> Sum/1
  [LExcSOL_MR] -> Sum3/1
  Saturation18/1 -> LExc/1
  Sum/1 -> Mux/1
  Mux1/1 -> Saturation1/1
  [RExcGAS_MG] -> Mux1/7
  [LExcRF_MG] -> Mux/4
  [LExcGLU_MG] -> Sum1/2
  [LExcTA_MR] -> Sum2/1
  [LExcTA_MG] -> Sum2/2
  [RExcVAS_MG] -> Mux1/5
  [LExcSOL_MG] -> Sum3/2
  [RExcHFL_MG] -> Sum4/2
  [RExcTA_MG] -> Sum6/2
  [RExcRF_MG] -> Mux1/4
  Sum3/1 -> Mux/8
  Mux/1 -> Saturation18/1
  [RExcSOL_MR] -> Sum7/1
  Sum1/1 -> Mux/2
  [LExcHFL_MG] -> Sum/2
  [RExcGLU_MR] -> Sum5/1
  Sum7/1 -> Mux1/8
  [LExcGAS_MG] -> Mux/7
  [RExcHFL_MR] -> Sum4/1
  [RExcSOL_MG] -> Sum7/2
  Saturation1/1 -> RExc/1
  Sum4/1 -> Mux1/1

== system nms_sim_2D_cost/Reflex Controller ==
  note: Control Parameters
  Constant10 : Constant  Value=TrCtrlPar
  Constant2 : Constant  Value=HLCtrlPar
  Constant5 : Constant  Value=StCtrlPar
  Constant9 : Constant  Value=SwCtrlPar
  Demux1 : Demux  Outputs=[1 1 3]
  Higher Control Layer (Supraspinal Control) : Subsystem
  Lower Control Layer (Spinal Cord) : Subsystem
      settings: PortSchema="{\"entries\":[{\"content\":{\"sides\":[{\"content\":{},\"type\":\"ConnectorPlacement.EquallySpacedRectSide\",\"uuid\":\"c3f799fd-f328-4fe6-8bbf-b27463c0ff63\"},{\"content\":{\"side\":\"RIGHT\"},\"type\":\"ConnectorPlacement.EquallySpacedRectSide\",\"uuid\":\"5c212595-efbc-4bb1-9e52-f061a0afb5ca\"},{\"content\":{\"side\":\"TOP\"},\"type\":\"ConnectorPlacement.EquallySpacedRectSide\",\"uuid\":\"e83b74d5-dc05-4e46-9f64-0074c32d6b2c\"},{\"content\":{\"connectorIds\":[\"Out1\",\"Out2\"],\"side\":\"BOTTOM\"},\"type\":\"ConnectorPlacement.EquallySpacedRectSide\",\"uuid\":\"cf249900-d8a7-48f1-916a-9e0c8ddf8fbd\"}]},\"type\":\"ConnectorPlacement.EquallySpacedConnector\",\"uuid\":\"c90eb79a-511f-4615-b41b-017cdb8cbfff\"}],\"packageUris\":[\"http://schema.mathworks.com/mf0/Connector/R2020b\"],\"version\":\"1.0\"}"
  LExc : Outport
  RExc : Outport  Port=2
  tag scope: StCtrlPar=global, SwCtrlPar=global, TrCtrlPar=global, alpha_par=global, leg_clr0=global, theta0=global
  wires:
  Constant5/1 -> [StCtrlPar]
  Constant10/1 -> [TrCtrlPar]
  Constant9/1 -> [SwCtrlPar]
  Demux1/3 -> [alpha_par]
  Demux1/1 -> [theta0]
  Demux1/2 -> [leg_clr0]
  Constant2/1 -> Demux1/1
  Lower Control Layer (Spinal Cord)/1(LExc) -> LExc/1
  Lower Control Layer (Spinal Cord)/2(RExc) -> RExc/1

== system nms_sim_2D_cost/Body Mechanics/LBall Contact ==
  note: 3D Ground Interaction Model
  Env : Inport
  2D Contact : Subsystem
  Demux : Demux  Outputs=2
  Demux2 : Demux  Outputs=[1 2 2]
  External Force and Torque : sm_lib/Forces and Torques/External Force and Torque  EnableForceX=on  EnableForceY=on  EnableForceZ=off  EnableForce=off  ForceResolutionFrame=World  EnableTorqueX=off  EnableTorqueY=off  EnableTorqueZ=off  EnableTorque=off  TorqueResolutionFrame=AttachedFrame
  Mux2 : Mux  Inputs=2
  Mux3 : Mux  Inputs=2
  PS-Simulink Converter : nesl_utility/PS-Simulink Converter  PhysicalDomain=network_engine_domain  SubClassName=ps_output  LeftPortType=input  RightPortType=output  PseudoPeriodic=off  Frequencies=[]  VectorFormat=1-D array  Unit=m  AffineConversion=off
  PS-Simulink Converter1 : nesl_utility/PS-Simulink Converter  PhysicalDomain=network_engine_domain  SubClassName=ps_output  LeftPortType=input  RightPortType=output  PseudoPeriodic=off  Frequencies=[]  VectorFormat=1-D array  Unit=m/s  AffineConversion=off
  PS-Simulink Converter2 : nesl_utility/PS-Simulink Converter  PhysicalDomain=network_engine_domain  SubClassName=ps_output  LeftPortType=input  RightPortType=output  PseudoPeriodic=off  Frequencies=[]  VectorFormat=1-D array  Unit=m  AffineConversion=off
  PS-Simulink Converter3 : nesl_utility/PS-Simulink Converter  PhysicalDomain=network_engine_domain  SubClassName=ps_output  LeftPortType=input  RightPortType=output  PseudoPeriodic=off  Frequencies=[]  VectorFormat=1-D array  Unit=m/s  AffineConversion=off
  Simulink-PS Converter : nesl_utility/Simulink-PS Converter  PhysicalDomain=network_engine_domain  SubClassName=ps_input  LeftPortType=input  RightPortType=output  PseudoPeriodic=off  Frequencies=[]  NoiseDistribution=none  NoiseParameters=[]  Unit=1  AffineConversion=off  FilteringAndDerivatives=zero  SimscapeFilterOrder=1  InputFilterTimeConstant=0.001  UdotUserProvided=1
  Simulink-PS Converter1 : nesl_utility/Simulink-PS Converter  PhysicalDomain=network_engine_domain  SubClassName=ps_input  LeftPortType=input  RightPortType=output  PseudoPeriodic=off  Frequencies=[]  NoiseDistribution=none  NoiseParameters=[]  Unit=1  AffineConversion=off  FilteringAndDerivatives=zero  SimscapeFilterOrder=1  InputFilterTimeConstant=0.001  UdotUserProvided=1
  Sum : Sum  Inputs=|+-
  Sum1 : Sum
  Transform Sensor : sm_lib/Frames and Transforms/Transform Sensor  MeasurementFrame=World  RotationSequence=XYX  SenseAngle=off  SenseAxis=off  SenseQ=off  SenseR=off  SenseRotationSequence=off  SenseOmegaX=off  SenseOmegaY=off  SenseOmegaZ=off  SenseOmega=off  SenseQDot=off  SenseRDot=off  SenseRotationSequenceDot=off  SenseAlphaX=off  SenseAlphaY=off  SenseAlphaZ=off  SenseAlpha=off  SenseQDDot=off  SenseRDDot=off  SenseX=on  SenseY=on  SenseZ=off  SenseXYZ=off  SenseRad=off  SenseAzim=off  SenseDist=off  SenseInc=off  SenseXDot=on  SenseYDot=on  SenseZDot=off  SenseXYZDot=off  SenseRadDot=off  SenseAzimDot=off  SenseDistDot=off  SenseIncDot=off  SenseXDDot=off  SenseYDDot=off  SenseZDDot=off  SenseXYZDDot=off  SenseRadDDot=off  SenseAzimDDot=off  SenseDistDDot=off  SenseIncDDot=off
  World Frame : sm_lib/Frames and Transforms/World Frame
  contact? : simulink/Logic and Bit Operations/Compare To Zero  relop=<=  OutDataTypeStr=boolean
  Foot : PMIOPort  Side=Left
  Cnt : Outport  VectorParamsAs1DForOutWhenUnconnected=off
  GRF [N N] : Outport  Port=2  VectorParamsAs1DForOutWhenUnconnected=off
  wires:
  contact?/1 -> Cnt/1, 2D Contact/Enable  "cnt"
  Env/1 -> Demux2/1
  2D Contact/1(FnVec [N N]) -> Sum1/1  "GRFn [N N]"
  2D Contact/2(FtVec [N N]) -> Sum1/2  "GRFt [N N]"
  Sum1/1 -> Demux/1, GRF [N N]/1
  Sum/1 -> contact?/1
  Demux2/1 -> Sum/2  "EnvHeight"
  Demux2/3 -> 2D Contact/2(nVec [m m])  "Normal Vector nVec"
  Mux2/1 -> 2D Contact/3(pVec [m m])
  Mux3/1 -> 2D Contact/4(vVec [m/s m/s])
  Demux2/2 -> 2D Contact/1(RefPt [m m])  "Reference Point RefPt"
  Demux/2 -> Simulink-PS Converter1/1
  Demux/1 -> Simulink-PS Converter/1
  PS-Simulink Converter3/1 -> Mux3/2
  PS-Simulink Converter2/1 -> Sum/1, Mux2/2
  PS-Simulink Converter1/1 -> Mux3/1
  PS-Simulink Converter/1 -> Mux2/1
  connections:
  External Force and Torque/RConn1 -- Transform Sensor/RConn1 -- Foot/RConn1
  External Force and Torque/LConn2 -- Simulink-PS Converter1/RConn1
  External Force and Torque/LConn1 -- Simulink-PS Converter/RConn1
  Transform Sensor/RConn2 -- PS-Simulink Converter/LConn1
  Transform Sensor/RConn4 -- PS-Simulink Converter1/LConn1
  Transform Sensor/RConn5 -- PS-Simulink Converter3/LConn1
  Transform Sensor/RConn3 -- PS-Simulink Converter2/LConn1
  Transform Sensor/LConn1 -- World Frame/RConn1

== system nms_sim_2D_cost/Body Mechanics/LHeel Contact ==
  note: 3D Ground Interaction Model
  Env : Inport
  2D Contact : Subsystem
  Demux : Demux  Outputs=2
  Demux2 : Demux  Outputs=[1 2 2]
  External Force and Torque : sm_lib/Forces and Torques/External Force and Torque  EnableForceX=on  EnableForceY=on  EnableForceZ=off  EnableForce=off  ForceResolutionFrame=World  EnableTorqueX=off  EnableTorqueY=off  EnableTorqueZ=off  EnableTorque=off  TorqueResolutionFrame=AttachedFrame
  Mux2 : Mux  Inputs=2
  Mux3 : Mux  Inputs=2
  PS-Simulink Converter : nesl_utility/PS-Simulink Converter  PhysicalDomain=network_engine_domain  SubClassName=ps_output  LeftPortType=input  RightPortType=output  PseudoPeriodic=off  Frequencies=[]  VectorFormat=1-D array  Unit=m  AffineConversion=off
  PS-Simulink Converter1 : nesl_utility/PS-Simulink Converter  PhysicalDomain=network_engine_domain  SubClassName=ps_output  LeftPortType=input  RightPortType=output  PseudoPeriodic=off  Frequencies=[]  VectorFormat=1-D array  Unit=m/s  AffineConversion=off
  PS-Simulink Converter2 : nesl_utility/PS-Simulink Converter  PhysicalDomain=network_engine_domain  SubClassName=ps_output  LeftPortType=input  RightPortType=output  PseudoPeriodic=off  Frequencies=[]  VectorFormat=1-D array  Unit=m  AffineConversion=off
  PS-Simulink Converter3 : nesl_utility/PS-Simulink Converter  PhysicalDomain=network_engine_domain  SubClassName=ps_output  LeftPortType=input  RightPortType=output  PseudoPeriodic=off  Frequencies=[]  VectorFormat=1-D array  Unit=m/s  AffineConversion=off
  Simulink-PS Converter : nesl_utility/Simulink-PS Converter  PhysicalDomain=network_engine_domain  SubClassName=ps_input  LeftPortType=input  RightPortType=output  PseudoPeriodic=off  Frequencies=[]  NoiseDistribution=none  NoiseParameters=[]  Unit=1  AffineConversion=off  FilteringAndDerivatives=zero  SimscapeFilterOrder=1  InputFilterTimeConstant=0.001  UdotUserProvided=1
  Simulink-PS Converter1 : nesl_utility/Simulink-PS Converter  PhysicalDomain=network_engine_domain  SubClassName=ps_input  LeftPortType=input  RightPortType=output  PseudoPeriodic=off  Frequencies=[]  NoiseDistribution=none  NoiseParameters=[]  Unit=1  AffineConversion=off  FilteringAndDerivatives=zero  SimscapeFilterOrder=1  InputFilterTimeConstant=0.001  UdotUserProvided=1
  Sum : Sum  Inputs=|+-
  Sum1 : Sum
  Transform Sensor : sm_lib/Frames and Transforms/Transform Sensor  MeasurementFrame=World  RotationSequence=XYX  SenseAngle=off  SenseAxis=off  SenseQ=off  SenseR=off  SenseRotationSequence=off  SenseOmegaX=off  SenseOmegaY=off  SenseOmegaZ=off  SenseOmega=off  SenseQDot=off  SenseRDot=off  SenseRotationSequenceDot=off  SenseAlphaX=off  SenseAlphaY=off  SenseAlphaZ=off  SenseAlpha=off  SenseQDDot=off  SenseRDDot=off  SenseX=on  SenseY=on  SenseZ=off  SenseXYZ=off  SenseRad=off  SenseAzim=off  SenseDist=off  SenseInc=off  SenseXDot=on  SenseYDot=on  SenseZDot=off  SenseXYZDot=off  SenseRadDot=off  SenseAzimDot=off  SenseDistDot=off  SenseIncDot=off  SenseXDDot=off  SenseYDDot=off  SenseZDDot=off  SenseXYZDDot=off  SenseRadDDot=off  SenseAzimDDot=off  SenseDistDDot=off  SenseIncDDot=off
  World Frame : sm_lib/Frames and Transforms/World Frame
  contact? : simulink/Logic and Bit Operations/Compare To Zero  relop=<=  OutDataTypeStr=boolean
  Foot : PMIOPort  Side=Left
  Cnt : Outport  VectorParamsAs1DForOutWhenUnconnected=off
  GRF [N N] : Outport  Port=2  VectorParamsAs1DForOutWhenUnconnected=off
  wires:
  contact?/1 -> Cnt/1, 2D Contact/Enable  "cnt"
  Env/1 -> Demux2/1
  2D Contact/1(FnVec [N N]) -> Sum1/1  "GRFn [N N]"
  2D Contact/2(FtVec [N N]) -> Sum1/2  "GRFt [N N]"
  Sum1/1 -> Demux/1, GRF [N N]/1
  Sum/1 -> contact?/1
  Demux2/1 -> Sum/2  "EnvHeight"
  Demux2/3 -> 2D Contact/2(nVec [m m])  "Normal Vector nVec"
  Mux2/1 -> 2D Contact/3(pVec [m m])
  Mux3/1 -> 2D Contact/4(vVec [m/s m/s])
  Demux2/2 -> 2D Contact/1(RefPt [m m])  "Reference Point RefPt"
  Demux/2 -> Simulink-PS Converter1/1
  Demux/1 -> Simulink-PS Converter/1
  PS-Simulink Converter3/1 -> Mux3/2
  PS-Simulink Converter2/1 -> Sum/1, Mux2/2
  PS-Simulink Converter1/1 -> Mux3/1
  PS-Simulink Converter/1 -> Mux2/1
  connections:
  Transform Sensor/RConn1 -- External Force and Torque/RConn1 -- Foot/RConn1
  External Force and Torque/LConn2 -- Simulink-PS Converter1/RConn1
  External Force and Torque/LConn1 -- Simulink-PS Converter/RConn1
  Transform Sensor/RConn2 -- PS-Simulink Converter/LConn1
  Transform Sensor/RConn4 -- PS-Simulink Converter1/LConn1
  Transform Sensor/RConn5 -- PS-Simulink Converter3/LConn1
  Transform Sensor/RConn3 -- PS-Simulink Converter2/LConn1
  Transform Sensor/LConn1 -- World Frame/RConn1

== system nms_sim_2D_cost/Body Mechanics/LLoad2 ==
  dxThigh [m] : Inport
  FB Gain1 : Gain  Gain=1/DeltaThRef  SaturateOnIntegerOverflow=on  OutDataTypeStr=Inherit: Same as input  ParamDataTypeStr=Inherit: Same as input
  Saturation11 : Saturate  UpperLimit=inf  LowerLimit=0  ZeroCross=off
  smooth2 : TransferFcn  Denominator=[0.02 1]
  LLoad [F] : Outport  VectorParamsAs1DForOutWhenUnconnected=off
  wires:
  Saturation11/1 -> FB Gain1/1
  smooth2/1 -> Saturation11/1
  FB Gain1/1 -> LLoad [F]/1
  dxThigh [m]/1 -> smooth2/1

== system nms_sim_2D_cost/Body Mechanics/LLoad3 ==
  dxThigh [m] : Inport
  FB Gain1 : Gain  Gain=1/DeltaThRef  SaturateOnIntegerOverflow=on  OutDataTypeStr=Inherit: Same as input  ParamDataTypeStr=Inherit: Same as input
  Saturation11 : Saturate  UpperLimit=inf  LowerLimit=0  ZeroCross=off
  smooth2 : TransferFcn  Denominator=[0.02 1]
  LLoad [F] : Outport  VectorParamsAs1DForOutWhenUnconnected=off
  wires:
  Saturation11/1 -> FB Gain1/1
  smooth2/1 -> Saturation11/1
  FB Gain1/1 -> LLoad [F]/1
  dxThigh [m]/1 -> smooth2/1
